simulink model "DemoSwc"  (R2024a)
settings: Solver=FixedStepDiscrete  StartTime=0.0  StopTime=10  FixedStep=0.01  RelTol=1e-3
model workspace (MAT data in the model file):
  FilterAlpha = Simulink.Parameter
  FilterAlpha.Value = 0.125
  FilterAlpha.Complexity = 'real'
  FilterAlpha.Dimensions = [1 1]
  FilterAlpha.DataType = 'single'
values from neighbouring files (symbols this model uses):
  FilterAlpha = 0.125    [DemoSwc_data.m]
undefined symbols (not defined in the file or in its folder): QLF_OK
libraries: simulink x2
settings Model: ParameterArgumentNames=FilterAlpha  Creator=danie  LastModifiedBy=danie
settings OptimizationCC: DefaultParameterBehavior=Inlined  EnhancedBackFolding=on  PassReuseOutputArgsAs=Individual arguments  ZeroExternalMemoryAtStartup=off  ZeroInternalMemoryAtStartup=off  OptimizeBlockOrder=speed  DifferentSizesBufferReuse=on  OptimizationCustomize=off  EfficientTunableParamExpr=on
settings DebuggingCC: ParameterTunabilityLossMsg=error
settings HardwareCC: ProdBitPerPointer=32  ProdBitPerSizeT=32  ProdBitPerPtrDiffT=32  ProdLargestAtomicInteger=Long  ProdLargestAtomicFloat=Double  ProdWordSize=32  ProdLongLongMode=on  ProdHWDeviceType=ARM Compatible->ARM Cortex-M
settings SFSimCC: MATLABDynamicMemAlloc=off
settings RTWCC: Description=AUTOSAR  SystemTargetFile=autosar.tlc  GenCodeOnly=on  GenerateMakefile=off  TemplateMakefile=ert_default_tmf  DataTypeReplacement=CDataTypesFixedWidth
settings CodeAppCC: ForceParamTrailComments=on  IgnoreCustomStorageClasses=off  MaxIdLength=63  OperatorAnnotations=on  SimulinkDataObjDesc=on  SFDataObjDesc=on  InsertBlockDesc=on
settings STFCustomTargetCC: MultiwordLength=256  ParMdlRefBuildCompliant=on  CompOptLevelCompliant=on  IncludeMdlTerminateFcn=off  CombineOutputUpdateFcns=on  SuppressErrorStatus=on  ERTCustomFileBanners=on  SupportNonFinite=off  SupportComplex=off  SupportContinuousTime=off  SupportNonInlinedSFcns=off  RemoveResetFunc=on  MATLABClassNameForMDSCustomization=Simulink.SoftwareTarget.ERTCustomization  AutosarCompliant=on  GRTInterface=off  LookupTableObjectStructAxisOrder=2,1,3,4,...  LUTObjectStructOrderEvenSpacing=Size,Table,Breakpoints  SystemTargetFile=autosar.tlc
settings ERTTargetCC: TargetLangStandard=C99 (ISO)  ConcurrentExecutionCompliant=off  IncludeMdlTerminateFcn=off  SuppressErrorStatus=on  SupportNonFinite=off  SupportComplex=off  ModelStepFunctionPrototypeControlCompliant=off  CPPClassGenCompliant=off  AutosarCompliant=on  LookupTableObjectStructAxisOrder=2,1,3,4,...  LUTObjectStructOrderEvenSpacing=Size,Table,Breakpoints  InlinedParameterPlacement=NonHierarchical  ERTCustomFileTemplate=example_file_process.tlc  BooleanTrueId=TRUE  BooleanFalseId=FALSE

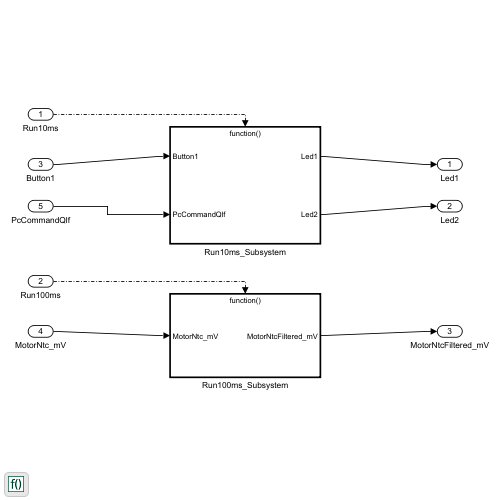
[thumbnail: Simulink's stored preview of the top-level diagram]
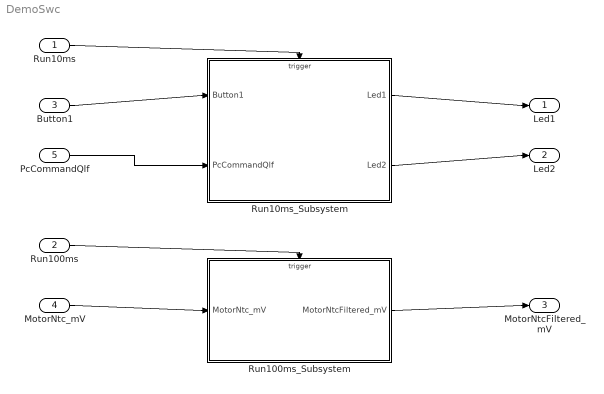
== system DemoSwc ==
  Run10ms : Inport  SampleTime=0.01  OutputFunctionCall=on
  Run100ms : Inport  Port=2  SampleTime=0.1  OutputFunctionCall=on
  Button1 : Inport  Port=3  OutDataTypeStr=boolean  PortDimensions=1
  MotorNtc_mV : Inport  Port=4  OutDataTypeStr=uint32  PortDimensions=1
  PcCommandQlf : Inport  Port=5  OutDataTypeStr=uint8  PortDimensions=1
  Run100ms_Subsystem : Subsystem  TreatAsAtomicUnit=on
  Run10ms_Subsystem : Subsystem  TreatAsAtomicUnit=on
  Led1 : Outport  OutDataTypeStr=boolean
  Led2 : Outport  Port=2  OutDataTypeStr=boolean
  MotorNtcFiltered_mV : Outport  Port=3  OutDataTypeStr=uint32
  wires:
  Run10ms/1 -> Run10ms_Subsystem/Trigger
  Button1/1 -> Run10ms_Subsystem/1(Button1)
  PcCommandQlf/1 -> Run10ms_Subsystem/2(PcCommandQlf)
  Run10ms_Subsystem/1(Led1) -> Led1/1
  Run10ms_Subsystem/2(Led2) -> Led2/1
  Run100ms/1 -> Run100ms_Subsystem/Trigger
  MotorNtc_mV/1 -> Run100ms_Subsystem/1(MotorNtc_mV)
  Run100ms_Subsystem/1(MotorNtcFiltered_mV) -> MotorNtcFiltered_mV/1

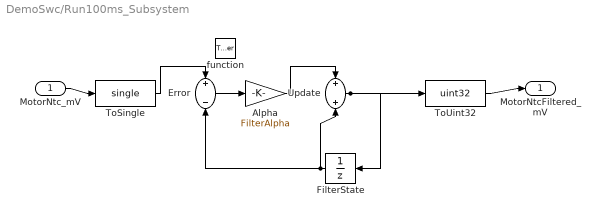
== system DemoSwc/Run100ms_Subsystem ==
  MotorNtc_mV : Inport
  function : TriggerPort  TriggerType=function-call  VariantControl=(inherit)
  Alpha : Gain  Gain=FilterAlpha
  Error : Sum  Inputs=+-
  FilterState : UnitDelay  SampleTime=-1  HasFrameUpgradeWarning=on
  ToSingle : DataTypeConversion  OutDataTypeStr=single  SaturateOnIntegerOverflow=off  RndMeth=Floor
  ToUint32 : DataTypeConversion  OutDataTypeStr=uint32  RndMeth=Nearest
  Update : Sum
  MotorNtcFiltered_mV : Outport
  wires:
  MotorNtc_mV/1 -> ToSingle/1
  ToSingle/1 -> Error/1
  Error/1 -> Alpha/1
  Alpha/1 -> Update/1
  Update/1 -> ToUint32/1, FilterState/1
  ToUint32/1 -> MotorNtcFiltered_mV/1
  FilterState/1 -> Error/2, Update/2

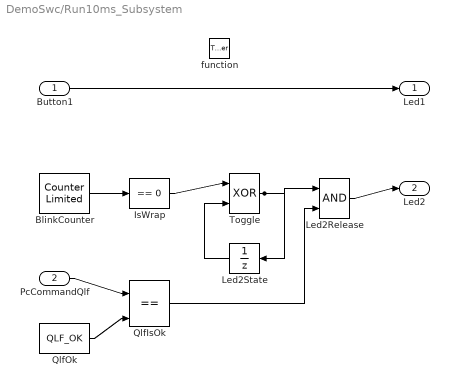
== system DemoSwc/Run10ms_Subsystem ==
  Button1 : Inport
  PcCommandQlf : Inport  Port=2
  function : TriggerPort  TriggerType=function-call  VariantControl=(inherit)
  BlinkCounter : simulink/Sources/Counter Limited  uplimit=49  tsamp=-1
  IsWrap : simulink/Logic and Bit Operations/Compare To Zero  relop===  OutDataTypeStr=boolean
  Led2Release : Logic  AllPortsSameDT=off  OutDataTypeStr=boolean
  Led2State : UnitDelay  InitialCondition=false  SampleTime=-1  HasFrameUpgradeWarning=on
  QlfIsOk : RelationalOperator  Operator===  OutDataTypeStr=boolean  RndMeth=Simplest  InputSameDT=off
  QlfOk : Constant  Value=QLF_OK  OutDataTypeStr=uint8
  Toggle : Logic  Operator=XOR  AllPortsSameDT=off  OutDataTypeStr=boolean
  Led1 : Outport
  Led2 : Outport  Port=2
  wires:
  Button1/1 -> Led1/1
  BlinkCounter/1 -> IsWrap/1
  IsWrap/1 -> Toggle/1
  Led2State/1 -> Toggle/2
  Toggle/1 -> Led2State/1, Led2Release/1
  PcCommandQlf/1 -> QlfIsOk/1
  QlfOk/1 -> QlfIsOk/2
  QlfIsOk/1 -> Led2Release/2
  Led2Release/1 -> Led2/1
